simulink model "lab3_dahlin"  (R2025b)
settings: Solver=ode45  StartTime=0.0  StopTime=40  MaxStep=0.05  RelTol=1e-3
settings Model: Creator=Nickolay  LastModifiedBy=Nickolay

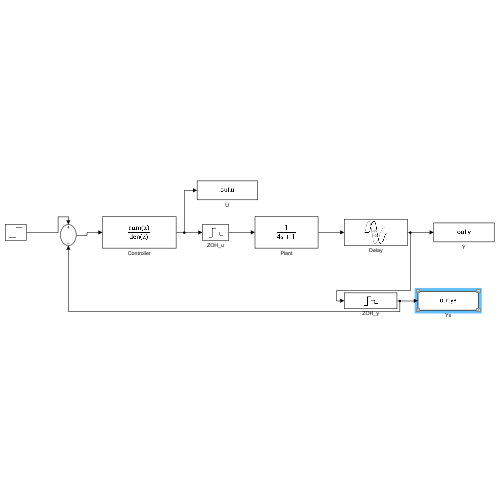
[thumbnail: Simulink's stored preview of the top-level diagram]
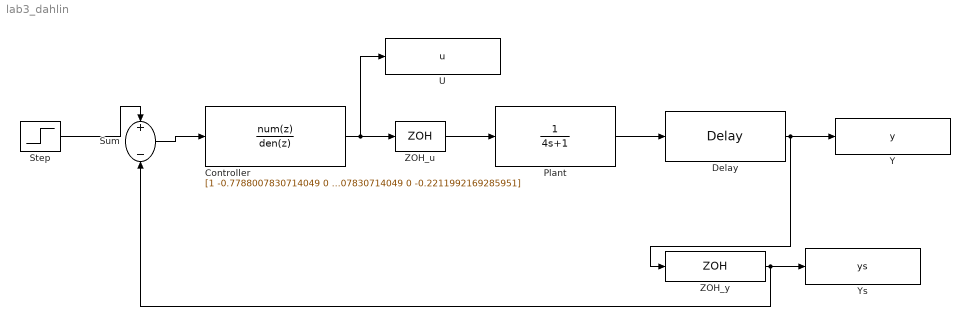
== system lab3_dahlin ==
  Controller : DiscreteTransferFcn  Numerator=[1 -0.7788007830714049 0 0]  Denominator=[1 -0.7788007830714049 0 -0.2211992169285951]  SampleTime=1
  Delay : TransportDelay  DelayTime=2
  Plant : TransferFcn  Denominator=[4 1]
  Step : Step  Time=0  SampleTime=0
  Sum : Sum  Inputs=+-
  U : ToWorkspace  VariableName=u  SaveFormat=Timeseries  SampleTime=-1
  Y : ToWorkspace  VariableName=y  SaveFormat=Timeseries  SampleTime=-1
  Ys : ToWorkspace  VariableName=ys  SaveFormat=Timeseries  SampleTime=-1
  ZOH_u : ZeroOrderHold
  ZOH_y : ZeroOrderHold
  wires:
  Step/1 -> Sum/1
  Sum/1 -> Controller/1
  Controller/1 -> ZOH_u/1, U/1
  ZOH_u/1 -> Plant/1
  Plant/1 -> Delay/1
  Delay/1 -> Y/1, ZOH_y/1
  ZOH_y/1 -> Sum/2, Ys/1
